simulink model "BSB_P_Regler_sim"  (R2026b)
settings: Solver=FixedStepAuto  StopTime=300  FixedStep=0.001  MinStep=0.05
libraries: slpidlib x1
settings Model: SimulationMode=accelerator  Creator=Enrico  LastModifiedBy=Enrico

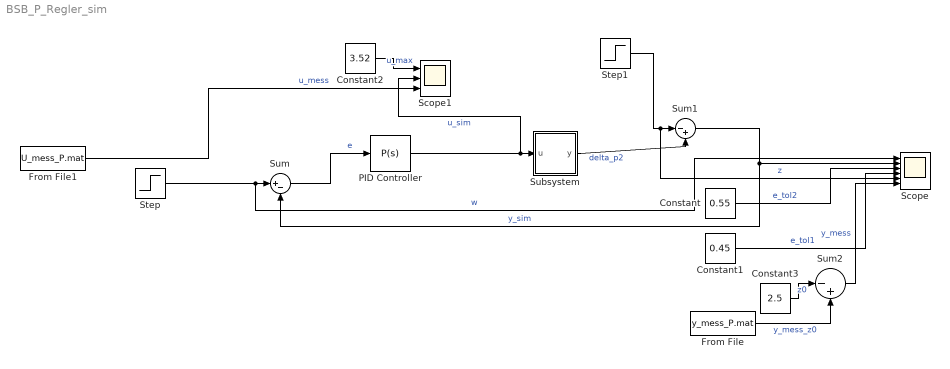
== system BSB_P_Regler_sim ==
  Constant : Constant  Value=0.55
  Constant1 : Constant  Value=0.45
  Constant2 : Constant  Value=3.52
  Constant3 : Constant  Value=2.5
  From File : FromFile  FileName=y_mess_P.mat  SampleTime=0
  From File1 : FromFile  FileName=U_mess_P.mat  SampleTime=0
  PID Controller : slpidlib/PID Controller  Controller=P  Form=Parallel  TimeDomain=Continuous-time  UseExternalTs=off  SampleTime=-1  IntegratorMethod=Forward Euler  FilterMethod=Forward Euler  ControllerParametersSource=internal  P=5.64  I=1  UseKiTs=off  D=0  UseExternalDerivativeSource=off  N=100  UseFilter=on  TunerSelectOption=Transfer Function Based (PID Tuner App)  InitialConditionSource=internal  InitialConditionForIntegrator=0  InitialConditionForFilter=0  DifferentiatorICPrevScaledInput=0  ExternalReset=none  TrackingMode=off  Kt=1  LimitOutput=off  SatLimitsSource=internal  UpperSaturationLimit=inf  LowerSaturationLimit=-inf  LinearizeAsGain=on  AntiWindupMode=none  Kb=1  LimitIntegrator=off  UpperIntegratorSaturationLimit=inf  LowerIntegratorSaturationLimit=-inf  POutMin=[]  POutMax=[]  IOutMin=[]  IOutMax=[]  DOutMin=[]  DOutMax=[]  NOutMin=[]  NOutMax=[]  SumOutMin=[]  SumOutMax=[]  SaturationOutMin=[]  SaturationOutMax=[]  PParamMin=[]  PParamMax=[]  IParamMin=[]  IParamMax=[]  DParamMin=[]  DParamMax=[]  NParamMin=[]  NParamMax=[]  KbParamMin=[]  KbParamMax=[]  KtParamMin=[]  KtParamMax=[]  KbOutMin=[]  KbOutMax=[]  KtOutMin=[]  KtOutMax=[]  IntegratorOutMin=[]  IntegratorOutMax=[]  FilterOutMin=[]  FilterOutMax=[]  SumI1OutMin=[]  SumI1OutMax=[]  SumI2OutMin=[]  SumI2OutMax=[]  SumI3OutMin=[]  SumI3OutMax=[]  SumI4OutMin=[]  SumI4OutMax=[]  SumDOutMin=[]  SumDOutMax=[]  DifferentiatorOutMin=[]  DifferentiatorOutMax=[]  FilterDiffOutCoefMin=[]  FilterDiffOutCoefMax=[]  ReciprocalOutMin=[]  ReciprocalOutMax=[]  SumDenOutMin=[]  SumDenOutMax=[]  SumNumOutMin=[]  SumNumOutMax=[]  DivideOutMin=[]  DivideOutMax=[]  UdiffTsProdOutMin=[]  UdiffTsProdOutMax=[]  NTsProdOutMin=[]  NTsProdOutMax=[]  UintegralTsProdOutMin=[]  UintegralTsProdOutMax=[]  UngainTsProdOutMin=[]  UngainTsProdOutMax=[]  ClampingZeroOutDataTypeStr=Inherit: Inherit via back propagation  ClampingZeroOutMin=[]  ClampingZeroOutMax=[]  FilterDenConstantOutDataTypeStr=Inherit: Inherit via back propagation  FilterDenConstantOutMin=[]  FilterDenConstantOutMax=[]  PCopyOutDataTypeStr=Inherit: Inherit via back propagation  PCopyOutMin=[]  PCopyOutMax=[]  NCopyOutDataTypeStr=Inherit: Inherit via back propagation  NCopyOutMin=[]  NCopyOutMax=[]  IntegratorContinuousStateAttributes=''  IntegratorStateMustResolveToSignalObject=off  IntegratorRTWStateStorageClass=Auto  FilterContinuousStateAttributes=''  FilterStateMustResolveToSignalObject=off  FilterRTWStateStorageClass=Auto  ParallelPVariant=InternalParameters  IdealPVariant=Disabled  IVariant=Disabled  DVariant=Disabled  IntegratorVariant=Disabled  SatVariant=Disabled  AWVariant=Disabled  PCopyVariant=Disabled  TRVariant=Disabled  FdbkBlocksVariant=Forward  IdealPFdbkVariant=Disabled  SatFdbkVariant=Disabled  DerivativeFilterVariant=Disabled  NVariant=Disabled  NCopyVariant=Disabled_SignalSpec  FilterICVariant=Disabled  IntegratorICVariant=Disabled  ExternalResetVariant=Disabled  TRSumVariant=Passthrough  SumFdbkVariant=Disabled  SumVariant=Passthrough_P  TsampFilterVariant=InternalTs  TsampNgainVariant=Passthrough  TsampIntegralVariant=Disabled_SignalSpec  ExternalSaturationOutDataTypeStr=Inherit: Same as second input  DerivativeSourceVariant=Disabled  PreIntVariant=InternalPreInt
  Scope : Scope  NumInputPorts=6
      settings: ActiveDisplayYMinimum=-0.19240818680736071  ActiveDisplayYMaximum=0.48340399400028722  DataLoggingMaxPoints=10000  DataLoggingDecimation=10
  Scope1 : Scope  NumInputPorts=3
      settings: ActiveDisplayYMinimum=1.1691467468790946  ActiveDisplayYMaximum=5.7562945738541664  DataLoggingMaxPoints=300000
  Step : Step  Time=100  FinalValue=0.5  SampleTime=0
  Step1 : Step  Time=200  FinalValue=0.5  SampleTime=0
  Subsystem : Subsystem  mask{Ks=0.54, Ta=1.5, Tb=10.5}
  Sum : Sum  Inputs=|+-
  Sum1 : Sum  Inputs=|-+
  Sum2 : Sum  Inputs=|-+
  wires:
  Step/1 -> Scope/1, Sum/1  "w"
  PID Controller/1 -> Scope1/2, Subsystem/1(u)  "u_sim"
  Sum/1 -> PID Controller/1  "e"
  Constant/1 -> Scope/3  "e_tol2"
  Constant1/1 -> Scope/4  "e_tol1"
  Step1/1 -> Scope/5, Sum1/1  "z"
  Subsystem/1(y) -> Sum1/2  "delta_p2"
  Sum1/1 -> Scope/2, Sum/2  "y_sim"
  Constant2/1 -> Scope1/1  "u_max"
  From File/1 -> Sum2/2  "y_mess_z0"
  Constant3/1 -> Sum2/1  "z0"
  Sum2/1 -> Scope/6  "y_mess"
  From File1/1 -> Scope1/3  "u_mess"

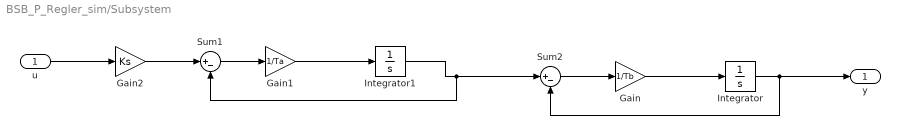
== system BSB_P_Regler_sim/Subsystem ==
  u : Inport
  Gain : Gain  Gain=1/Tb
  Gain1 : Gain  Gain=1/Ta
  Gain2 : Gain  Gain=Ks
  Integrator : Integrator
  Integrator1 : Integrator
  Sum1 : Sum  Inputs=|+-
  Sum2 : Sum  Inputs=|+-
  y : Outport
  wires:
  Integrator/1 -> y/1, Sum2/2
  u/1 -> Gain2/1
  Gain1/1 -> Integrator1/1
  Sum1/1 -> Gain1/1
  Gain/1 -> Integrator/1
  Integrator1/1 -> Sum2/1, Sum1/2
  Sum2/1 -> Gain/1
  Gain2/1 -> Sum1/1
